simulink model "THSDemo"  (R2023a)
settings: Solver=ode4  StartTime=210  StopTime=260  FixedStep=0.002  RelTol=1e-3
InitFcn:
  |  T_c = 0.002;
undefined symbols (not defined in the file or in its folder): DiscIntNeverNeededParam, Discrete, magnitude, Time
libraries: simulink x23, simulink_extras x8, sharedtransform x3, ctrlSharedLib x2, aerolibconvert2 x1, aerolibtransform2 x1, dspstat3 x1, dspsolvers x1
(part 2 of 2)

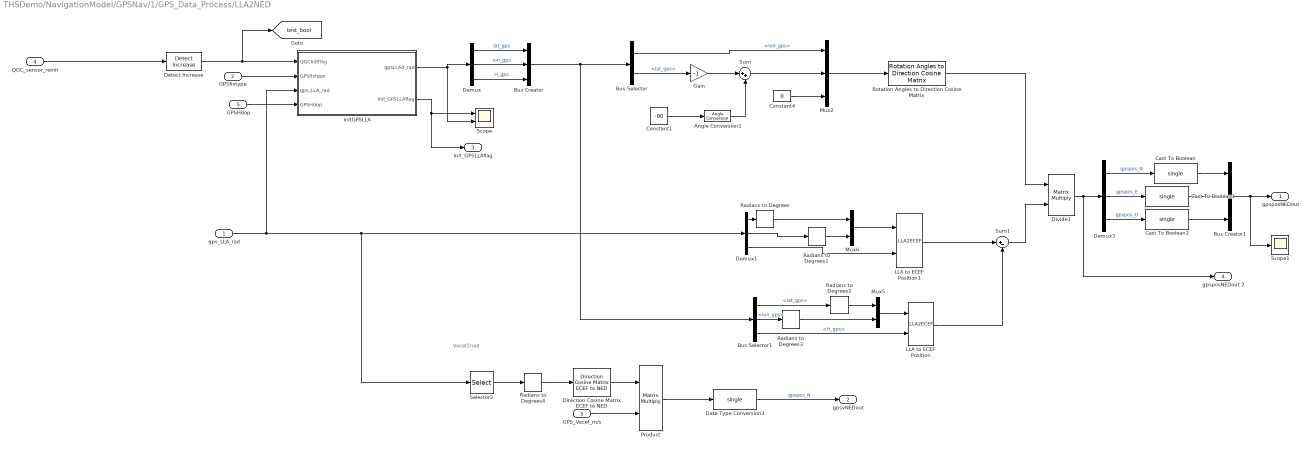
== system THSDemo/NavigationModel/GPSNav/1/GPS_Data_Process/LLA2NED ==
  note: Vecef2ned
  gps_LLA_rad : Inport
  GPSfixtype : Inport  Port=2
  GPS_Vecef_m/s : Inport  Port=3
  QGC_sensor_reinit : Inport  Port=4
  GPSHdop : Inport  Port=5
  Angle Conversion1 : aerolibconvert2/Angle Conversion  IU=deg  OU=rad
  Bus Creator : BusCreator  Inputs=3
  Bus Creator1 : BusCreator  Inputs=3
  Bus Selector : BusSelector  OutputSignals=lon_gps,lat_gps
  Bus Selector1 : BusSelector  OutputSignals=lat_gps,lon_gps,H_gps
  Cast To Boolean : DataTypeConversion  OutDataTypeStr=single  SaturateOnIntegerOverflow=off  RndMeth=Floor
  Cast To Boolean1 : DataTypeConversion  OutDataTypeStr=single  SaturateOnIntegerOverflow=off  RndMeth=Floor
  Cast To Boolean2 : DataTypeConversion  OutDataTypeStr=single  SaturateOnIntegerOverflow=off  RndMeth=Floor
  Constant1 : Constant  Value=-90
  Constant4 : Constant  Value=0
  Data Type Conversion3 : DataTypeConversion  OutDataTypeStr=single  SaturateOnIntegerOverflow=off  RndMeth=Floor
  Demux : Demux  Outputs=3
  Demux1 : Demux  Outputs=3
  Demux3 : Demux  Outputs=3
  Detect Increase : simulink/Logic and Bit Operations/Detect Increase  vinit=0.0  OutDataTypeStr=boolean
  Direction Cosine Matrix ECEF to NED : aerolibtransform2/Direction Cosine Matrix ECEF to NED
  Divide1 : Product  Inputs=**  Multiplication=Matrix(*)
  Gain : Gain  Gain=-1
  LLA to ECEF Position : LLA2ECEF  R=6378137
  LLA to ECEF Position1 : LLA2ECEF  R=6378137
  Mux2 : Mux  Inputs=3
  Mux5 : Mux  Inputs=2
  Mux6 : Mux  Inputs=2
  Product : Product  Multiplication=Matrix(*)
  Radians to Degrees{,1..4} (5 alike) : simulink_extras/Transformations/Radians to Degrees
  Rotation Angles to Direction Cosine Matrix : sharedtransform/Rotation Angles to Direction Cosine Matrix  rotationOrder=ZYX  aMode=aMode
  Scope : Scope  NumInputPorts=2
  Scope1 : Scope
  Selector2 : Selector  InputPortWidth=3  IndexOptions=Index vector (dialog)  Indices=[1 2]  OutputSizes=1
  Sum : Sum  Inputs=|++
  Sum1 : Sum  Inputs=|+-
  initGPSLLA : MATLAB Function  TreatAsAtomicUnit=on
  "gpsposNEDout " : Outport
  gpsvNEDout : Outport  Port=2
  init_GPSLLAflag : Outport  Port=3
  gpsposNEDout 2 : Outport  Port=4
  tag scope: test_bool=global
  wires:
  GPSfixtype/1 -> initGPSLLA/2(GPSfixtype)
  Bus Creator1/1 -> Scope1/1, "gpsposNEDout "/1
  Demux3/3 -> Cast To Boolean2/1  "gpspos_D"
  Demux3/2 -> Cast To Boolean1/1  "gpspos_E"
  Demux3/1 -> Cast To Boolean/1  "gpspos_N"
  Bus Creator/1 -> Bus Selector/1, Bus Selector1/1
  Demux/3 -> Bus Creator/3  "H_gps"
  Demux/2 -> Bus Creator/2  "lon_gps"
  Demux/1 -> Bus Creator/1  "lat_gps"
  Demux1/3 -> LLA to ECEF Position1/2
  Mux6/1 -> LLA to ECEF Position1/1
  Mux5/1 -> LLA to ECEF Position/1
  Gain/1 -> Sum/1
  LLA to ECEF Position1/1 -> Sum1/1
  Constant4/1 -> Mux2/3
  Sum1/1 -> Divide1/2
  Divide1/1 -> gpsposNEDout 2/1, Demux3/1
  Demux1/1 -> Radians to Degrees/1
  Mux2/1 -> Rotation Angles to Direction Cosine Matrix/1
  Rotation Angles to Direction Cosine Matrix/1 -> Divide1/1
  Constant1/1 -> Angle Conversion1/1
  LLA to ECEF Position/1 -> Sum1/2
  Demux1/2 -> Radians to Degrees1/1
  Sum/1 -> Mux2/2
  Bus Selector/2 -> Gain/1  "<lat_gps>"
  Bus Selector/1 -> Mux2/1  "<lon_gps>"
  Bus Selector1/1 -> Radians to Degrees2/1  "<lat_gps>"
  Bus Selector1/2 -> Radians to Degrees3/1  "<lon_gps>"
  Bus Selector1/3 -> LLA to ECEF Position/2  "<H_gps>"
  gps_LLA_rad/1 -> initGPSLLA/3(gps_LLA_rad), Selector2/1, Demux1/1
  Radians to Degrees/1 -> Mux6/1
  Radians to Degrees1/1 -> Mux6/2
  Angle Conversion1/1 -> Sum/2
  Radians to Degrees2/1 -> Mux5/1
  Radians to Degrees3/1 -> Mux5/2
  GPS_Vecef_m/s/1 -> Product/2
  Direction Cosine Matrix ECEF to NED/1 -> Product/1
  Selector2/1 -> Radians to Degrees4/1
  Radians to Degrees4/1 -> Direction Cosine Matrix ECEF to NED/1
  Data Type Conversion3/1 -> gpsvNEDout/1  "gpspos_N"
  Detect Increase/1 -> [test_bool], initGPSLLA/1(QGCinitflag)
  initGPSLLA/1(gpsLLA0_rad) -> Demux/1, Scope/2
  initGPSLLA/2(init_GPSLLAflag) -> init_GPSLLAflag/1, Scope/1
  GPSHdop/1 -> initGPSLLA/4(GPSHdop)
  Cast To Boolean/1 -> Bus Creator1/1
  Cast To Boolean1/1 -> Bus Creator1/2
  Cast To Boolean2/1 -> Bus Creator1/3
  QGC_sensor_reinit/1 -> Detect Increase/1
  Product/1 -> Data Type Conversion3/1

== system THSDemo/NavigationModel/GPSNav/1/GPS_Data_Process/TD_baro ==
  H_baro : Inport
  Constant1 : Constant  Value=0.002  OutDataTypeStr=double
  Constant3 : Constant  Value=0.23  OutDataTypeStr=double
  Constant4 : Constant  Value=900  OutDataTypeStr=single
  Data Type Conversion : DataTypeConversion  OutDataTypeStr=single  SaturateOnIntegerOverflow=off  RndMeth=Floor
  Data Type Conversion1 : DataTypeConversion  OutDataTypeStr=single  SaturateOnIntegerOverflow=off  RndMeth=Floor
  Data Type Conversion5 : DataTypeConversion  OutDataTypeStr=single  SaturateOnIntegerOverflow=off  RndMeth=Floor
  Delay1 : Delay  DelayLength=1  InitialConditionSource=Input port
      settings: InputPortMap=u0,p4
  MATLAB Function2 : MATLAB Function  TreatAsAtomicUnit=on
  Memory : Memory  InheritSampleTime=on
  Scope : Scope  NumInputPorts=3
  vH_baro_TD : Outport
  H_baro_TD : Outport  Port=2
  wires:
  Delay1/1 -> H_baro_TD/1, Scope/3, MATLAB Function2/3("u1 ")
  H_baro/1 -> Data Type Conversion5/1
  Memory/1 -> MATLAB Function2/4("u2 "), vH_baro_TD/1, Scope/2
  Constant3/1 -> Data Type Conversion1/1
  Constant4/1 -> MATLAB Function2/6(r)
  MATLAB Function2/1(u1) -> Delay1/1
  MATLAB Function2/2(u2) -> Memory/1
  Data Type Conversion5/1 -> Scope/1, Delay1/2, MATLAB Function2/2(u0)
  Constant1/1 -> Data Type Conversion/1
  Data Type Conversion/1 -> MATLAB Function2/1(T)
  Data Type Conversion1/1 -> MATLAB Function2/5(h)

== system THSDemo/NavigationModel/GPSNav/1/GPS_Data_Process/TD_baro1 ==
  H_baro : Inport
  Constant1 : Constant  Value=0.002  OutDataTypeStr=double
  Constant3 : Constant  Value=0.23  OutDataTypeStr=double
  Constant4 : Constant  Value=900  OutDataTypeStr=single
  Data Type Conversion : DataTypeConversion  OutDataTypeStr=single  SaturateOnIntegerOverflow=off  RndMeth=Floor
  Data Type Conversion1 : DataTypeConversion  OutDataTypeStr=single  SaturateOnIntegerOverflow=off  RndMeth=Floor
  Data Type Conversion5 : DataTypeConversion  OutDataTypeStr=single  SaturateOnIntegerOverflow=off  RndMeth=Floor
  Delay1 : Delay  DelayLength=1  InitialConditionSource=Input port
      settings: InputPortMap=u0,p4
  MATLAB Function2 : MATLAB Function  TreatAsAtomicUnit=on
  Memory : Memory  InheritSampleTime=on
  Scope : Scope  NumInputPorts=3
  vH_baro_TD : Outport
  H_baro_TD : Outport  Port=2
  wires:
  Data Type Conversion5/1 -> MATLAB Function2/2(u0), Delay1/2, Scope/1
  MATLAB Function2/2(u2) -> Memory/1
  MATLAB Function2/1(u1) -> Delay1/1
  Constant4/1 -> MATLAB Function2/6(r)
  Constant1/1 -> Data Type Conversion/1
  Constant3/1 -> Data Type Conversion1/1
  Memory/1 -> Scope/2, vH_baro_TD/1, MATLAB Function2/4("u2 ")
  H_baro/1 -> Data Type Conversion5/1
  Delay1/1 -> MATLAB Function2/3("u1 "), Scope/3, H_baro_TD/1
  Data Type Conversion/1 -> MATLAB Function2/1(T)
  Data Type Conversion1/1 -> MATLAB Function2/5(h)

== system THSDemo/NavigationModel/GPSNav/1/GPS_Data_Process/heading_GPS ==
  Vned : Inport
  Atan2 : Trigonometry  Operator=atan2
  Compare To Constant : simulink/Logic and Bit Operations/Compare To Constant  relop=>  const=0.8  OutDataTypeStr=boolean
  Data Type Conversion : DataTypeConversion  OutDataTypeStr=double  SaturateOnIntegerOverflow=off  RndMeth=Floor
  Math Function : Math  Operator=magnitude^2  SignedPower=on
  Moving Average1 : dspstat3/Moving Average  Commented=on  Method=Sliding window  ForgettingFactorPort=off  SpecifyWindowLength=on  WindowLength=10  OverlapLength=9  AllowArbitraryInputLength=off  ForgettingFactor=0.9  SimulateUsing=Code generation
  Rate Transition : RateTransition  OutPortSampleTime=1
  Scope : Scope  NumInputPorts=2
  Scope1 : Scope
  Selector2 : Selector  InputPortWidth=3  IndexOptions=Index vector (dialog)  Indices=[2]  OutputSizes=1
  Selector3 : Selector  InputPortWidth=3  IndexOptions=Index vector (dialog)  Indices=[1]  OutputSizes=1
  Selector4 : Selector  InputPortWidth=3  IndexOptions=Index vector (dialog)  Indices=[1 2]  OutputSizes=1
  Sqrt : Sqrt
  Sum of Elements : Sum  Inputs=+
  heading_GPS_rad : Outport
  heading_GPS_valid : Outport  Port=2
  wires:
  Selector2/1 -> Atan2/1
  Math Function/1 -> Sum of Elements/1
  Vned/1 -> Selector2/1, Selector4/1, Selector3/1
  Selector3/1 -> Atan2/2
  Sum of Elements/1 -> Sqrt/1
  Selector4/1 -> Math Function/1
  Sqrt/1 -> Data Type Conversion/1
  Compare To Constant/1 -> Scope1/1, heading_GPS_valid/1
  Rate Transition/1 -> Scope/1, Scope/2, heading_GPS_rad/1
  Atan2/1 -> Rate Transition/1
  Data Type Conversion/1 -> Compare To Constant/1

== system THSDemo/NavigationModel/GPSNav/1/Translation_estimate/Subsystem ==
  vxy : Inport
  pxy_GPS : Inport  Port=2
  GPSv_enable : Inport  Port=3
  QGC_init : Inport  Port=4
  DOP : Inport  Port=5
  Add : Sum  Inputs=+-
  Add1 : Sum  Inputs=++-
  Compare To Constant : simulink/Logic and Bit Operations/Compare To Constant  relop=<=  const=3  OutDataTypeStr=boolean
  Delay : Delay  DelayLength=1  InitialCondition=[0;0;]  ExternalReset=Rising
      settings: InputPortMap=u0,r5
  Detect Change : simulink/Logic and Bit Operations/Detect Change  vinit=0  OutDataTypeStr=boolean
  Gain : Gain  Gain=0.002
  Kalman Filter : ctrlSharedLib/Kalman Filter  TimeDomain=Discrete-Time  UseCurrentEstimator=on  ModelSource=Individual A, B, C, D matrices  ModelSourceVariable=ss(0.95,1,1,0,1)  A=[0.1,0;0,0.1]  B=eye(2)  C=eye(2)  D=0  NumberOfStates=1  NumberOfInputs=1  NumberOfOutputs=1  InitialEstimateSource=Dialog  X0=0  P0=10  UseK=off  UseGH=off  NumberOfProcessNoiseInputs=1  G=1  TimeInvariantG=on  H=0  TimeInvariantH=on  Q=diag([0.1;0.1])  TimeInvariantQ=on  R=diag([0.8;0.8])  TimeInvariantR=on  N=0  TimeInvariantN=on  AddInputPort=off  AddEnablePort=on  ExternalReset=Rising  OutputEstimatedY=off  OutputP=off  Ts=-1
  Logical Operator : Logic  AllPortsSameDT=off  OutDataTypeStr=boolean
  Memory : Memory
  Product : Product  OutDataTypeStr=double
  QGC_init1 : InportShadow  Port=4
  Rate Transition1 : RateTransition  OutPortSampleTime=0.002
  Rate Transition2 : RateTransition  OutPortSampleTime=0.002
  Rate Transition3 : RateTransition  OutPortSampleTime=0.002
  Scope7 : Scope
  Selector : Selector  InputPortWidth=2  IndexOptions=Index vector (dialog)  Indices=[1]  OutputSizes=1
  pxy_est : Outport
  wires:
  Gain/1 -> Add1/1
  Delay/1 -> Add1/2
  Kalman Filter/1 -> Product/1
  pxy_GPS/1 -> Selector/1, Add/2
  Selector/1 -> Detect Change/1
  Product/1 -> Memory/1
  Logical Operator/1 -> Product/2, Rate Transition2/1
  Rate Transition2/1 -> Scope7/1, Kalman Filter/2
  Rate Transition1/1 -> Kalman Filter/1
  Memory/1 -> Add1/3
  Add/1 -> Rate Transition1/1
  vxy/1 -> Gain/1
  Add1/1 -> Add/1, Delay/1, pxy_est/1
  QGC_init/1 -> Rate Transition3/1
  Rate Transition3/1 -> Kalman Filter/3
  DOP/1 -> Compare To Constant/1
  Compare To Constant/1 -> Logical Operator/2
  QGC_init1/1 -> Delay/2
  GPSv_enable/1 -> Logical Operator/1

== system THSDemo/NavigationModel/GPSNav/1/Translation_estimate/Subsystem2 ==
  axy : Inport
  vxy_GPS : Inport  Port=2
  QGC_init : Inport  Port=3
  DOP : Inport  Port=4
  Add : Sum  Inputs=+-
  Add1 : Sum  Inputs=++-
  Compare To Constant : simulink/Logic and Bit Operations/Compare To Constant  relop=<=  const=3  OutDataTypeStr=boolean
  Delay : Delay  DelayLength=1  ExternalReset=Rising
      settings: InputPortMap=u0,r5
  Detect Change : simulink/Logic and Bit Operations/Detect Change  vinit=0  OutDataTypeStr=boolean
  Gain : Gain  Gain=0.002
  Kalman Filter : ctrlSharedLib/Kalman Filter  TimeDomain=Discrete-Time  UseCurrentEstimator=on  ModelSource=Individual A, B, C, D matrices  ModelSourceVariable=ss(0.95,1,1,0,1)  A=[0.6,0;0,0.6]  B=eye(2)  C=eye(2)  D=0  NumberOfStates=1  NumberOfInputs=1  NumberOfOutputs=1  InitialEstimateSource=Dialog  X0=0  P0=10  UseK=off  UseGH=off  NumberOfProcessNoiseInputs=1  G=1  TimeInvariantG=on  H=0  TimeInvariantH=on  Q=diag([0.1;0.1])  TimeInvariantQ=on  R=diag([0.6;0.6])  TimeInvariantR=on  N=0  TimeInvariantN=on  AddInputPort=off  AddEnablePort=on  ExternalReset=Rising  OutputEstimatedY=off  OutputP=off  Ts=-1
  Logical Operator : Logic  AllPortsSameDT=off  OutDataTypeStr=boolean
  Memory : Memory
  Product : Product  OutDataTypeStr=double
  Rate Transition1 : RateTransition  OutPortSampleTime=0.002
  Rate Transition2 : RateTransition  OutPortSampleTime=0.002
  Rate Transition3 : RateTransition  OutPortSampleTime=0.002
  Scope : Scope  NumInputPorts=2
  Scope7 : Scope
  Selector : Selector  InputPortWidth=2  IndexOptions=Index vector (dialog)  Indices=[1]  OutputSizes=1
  vxy_est : Outport
  GPSv_enable : Outport  Port=2
  wires:
  Compare To Constant/1 -> Logical Operator/2
  DOP/1 -> Compare To Constant/1
  Detect Change/1 -> Logical Operator/1
  Rate Transition3/1 -> Kalman Filter/3
  QGC_init/1 -> Delay/2, Rate Transition3/1
  Add1/1 -> Delay/1, vxy_est/1, Scope/1, Add/1
  Add/1 -> Rate Transition1/1
  Memory/1 -> Add1/3
  Rate Transition1/1 -> Kalman Filter/1
  Rate Transition2/1 -> Scope7/1, Kalman Filter/2
  Logical Operator/1 -> GPSv_enable/1, Rate Transition2/1, Product/2
  Product/1 -> Memory/1
  Selector/1 -> Detect Change/1
  vxy_GPS/1 -> Selector/1, Add/2, Scope/2
  Kalman Filter/1 -> Product/1
  Gain/1 -> Add1/1
  axy/1 -> Gain/1
  Delay/1 -> Add1/2

== system THSDemo/NavigationModel/GPSNav/1/Translation_estimate/V_Horizontal_estimation1 ==
  note: 0530改：
      | 加入GPStype限制
  An : Inport
  vn_gps : Inport  Port=2
  ve_gps : Inport  Port=3
  fixtype_gps : Inport  Port=4
  QGC_init : Inport  Port=5
  Add : Sum  Inputs=+-
  Compare To Constant : simulink/Logic and Bit Operations/Compare To Constant  relop=>=  const=3  OutDataTypeStr=boolean
  Delay : Delay  DelayLength=1
  Detect Change : simulink/Logic and Bit Operations/Detect Change  vinit=0  OutDataTypeStr=boolean
  Integrator_V_Horizontal : Subsystem
  Logical Operator : Logic  AllPortsSameDT=off  OutDataTypeStr=boolean
  Mux : Mux  Inputs=2
  Rxy_kalman filter1 : Subsystem  mask{F=diag([-0.1,-0.1,-0.002,-0.002]), H=[1,0,-1,0;0,1,0,-1], Q=diag([1,1,0.1,0.1]), R=diag([0.001,0.001]), P0=diag([0.8,0.8,0.2,0.2])}
      mask prompts: F "状态转移矩阵：F"; H "观测转移矩阵：H"; Q "预测噪声协方差矩阵：Q"; R "量测噪声协方差矩阵：R"; P0 "初始协方差矩阵：P0"
      mask DialogControl DescTextVar Prompt: Kalman Filter
  Scope : Scope  NumInputPorts=2
  Scope1 : Scope
  Selector : Selector  InputPortWidth=4  IndexOptions=Index vector (dialog)  Indices=[1 2]  OutputSizes=1
  vxy_estimout : Outport
  GPS_v_enable : Outport  Port=2
  wires:
  QGC_init/1 -> Integrator_V_Horizontal/3(QGC_init)
  Delay/1 -> Selector/1, Rxy_kalman filter1/1(X)
  Selector/1 -> Integrator_V_Horizontal/2(dv)
  vn_gps/1 -> Integrator_V_Horizontal/4(vn_gps), Mux/1, Detect Change/1
  Mux/1 -> Scope/2, Add/2
  ve_gps/1 -> Integrator_V_Horizontal/5(ve_gps), Mux/2
  Rxy_kalman filter1/1(XOut) -> Delay/1
  Integrator_V_Horizontal/1(V_n&e) -> Add/1, vxy_estimout/1, Scope/1
  Add/1 -> Rxy_kalman filter1/2(Z)
  An/1 -> Integrator_V_Horizontal/1(An)
  fixtype_gps/1 -> Compare To Constant/1
  Detect Change/1 -> Logical Operator/1
  Compare To Constant/1 -> Logical Operator/2, Scope1/1, GPS_v_enable/1, Rxy_kalman filter1/3(Enable), Integrator_V_Horizontal/6(GPSenable)

== system THSDemo/NavigationModel/GPSNav/1/Translation_estimate/translate to N ==
  Cbn : Inport
  accl_ned : Inport  Port=2
  Product : Product  Multiplication=Matrix(*)
  Selector : Selector  InputPortWidth=3  IndexOptions=Index vector (dialog)  Indices=[1 2]  OutputSizes=1
  accel_Horizontal_predict : Outport
  wires:
  Selector/1 -> accel_Horizontal_predict/1
  Product/1 -> Selector/1
  Cbn/1 -> Product/1
  accl_ned/1 -> Product/2

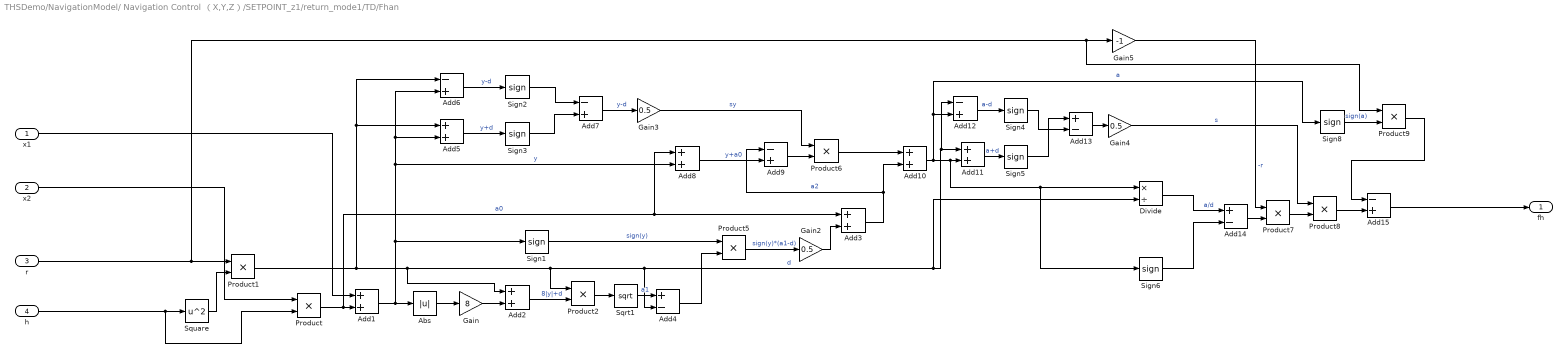
== system THSDemo/NavigationModel/ Navigation Control （X,Y,Z）/SETPOINT_z1/return_mode1/TD/Fhan ==
  x1 : Inport
  x2 : Inport  Port=2
  r : Inport  Port=3
  h : Inport  Port=4
  Abs : Abs  SaturateOnIntegerOverflow=off
  Add{1..3,5,8,10..11} (7 alike) : Sum
  Add{6..7,9,12,15} (5 alike) : Sum  Inputs=-+
  Add13 : Sum  Inputs=+-
  Add14 : Sum  Inputs=+-
  Add4 : Sum  Inputs=+-
  Divide : Product  Inputs=*/
  Gain : Gain  Gain=8
  Gain2 : Gain  Gain=0.5
  Gain3 : Gain  Gain=0.5
  Gain4 : Gain  Gain=0.5
  Gain5 : Gain  Gain=-1
  Product{,1..2,5..9} (8 alike) : Product
  Sign{1..6,8} (7 alike) : Signum
  Sqrt1 : Sqrt
  Square : Math  Operator=square  SignedPower=on
  fh : Outport
  wires:
  Add1/1 -> Add8/2, Add6/2, Add5/2, Sign1/1, Abs/1  "y"
  Product1/1 -> Add6/1, Add5/1, Divide/2, Add12/1, Add11/1, Add4/2, Product2/1, Add2/1  "d"
  Add5/1 -> Sign3/1  "y+d"
  Sign4/1 -> Add13/2
  Add9/1 -> Product6/2
  Product5/1 -> Gain2/1  "sign(y)*(a1-d)"
  Gain3/1 -> Product6/1  "sy"
  Product/1 -> Add8/1, Add3/1, Add1/2  "a0"
  Product6/1 -> Add10/1
  Add7/1 -> Gain3/1  "y-d"
  Sign8/1 -> Product9/2  "sign(a)"
  Sign3/1 -> Add7/2
  Add2/1 -> Product2/2  "8|y|+d"
  r/1 -> Product9/1, Gain5/1, Product1/1
  Add10/1 -> Sign6/1, Divide/1, Add11/2, Add12/2, Sign8/1  "a"
  Product2/1 -> Sqrt1/1
  Sign5/1 -> Add13/1
  Abs/1 -> Gain/1
  Divide/1 -> Add14/1  "a/d"
  Gain2/1 -> Add3/2
  Gain/1 -> Add2/2
  Add13/1 -> Gain4/1
  Add14/1 -> Product7/2
  Add3/1 -> Add10/2, Add9/1  "a2"
  Add12/1 -> Sign4/1  "a-d"
  Gain4/1 -> Product8/1  "s"
  Product8/1 -> Add15/2
  h/1 -> Product/2, Square/1
  Square/1 -> Product1/2
  Add8/1 -> Add9/2  "y+a0"
  Sign6/1 -> Add14/2
  Add11/1 -> Sign5/1  "a+d"
  Sign2/1 -> Add7/1
  Sqrt1/1 -> Add4/1  "a1"
  Product9/1 -> Add15/1
  Add4/1 -> Product5/2
  Add6/1 -> Sign2/1  "y-d"
  Sign1/1 -> Product5/1  "sign(y)"
  Product7/1 -> Product8/2
  Gain5/1 -> Product7/1  "-r"
  x1/1 -> Add1/1
  x2/1 -> Product/1
  Add15/1 -> fh/1

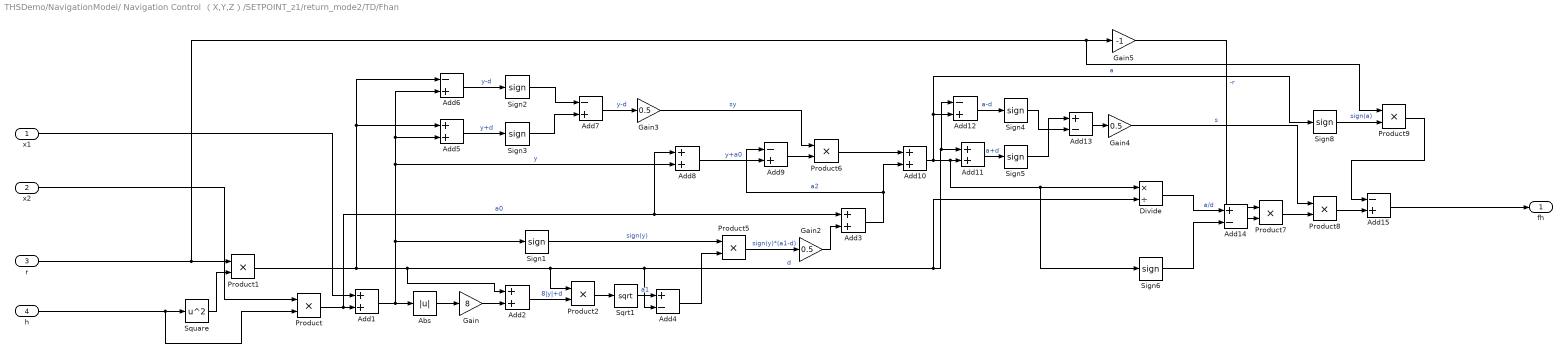
== system THSDemo/NavigationModel/ Navigation Control （X,Y,Z）/SETPOINT_z1/return_mode2/TD/Fhan ==
  x1 : Inport
  x2 : Inport  Port=2
  r : Inport  Port=3
  h : Inport  Port=4
  Abs : Abs  SaturateOnIntegerOverflow=off
  Add{1..3,5,8,10..11} (7 alike) : Sum
  Add{6..7,9,12,15} (5 alike) : Sum  Inputs=-+
  Add13 : Sum  Inputs=+-
  Add14 : Sum  Inputs=+-
  Add4 : Sum  Inputs=+-
  Divide : Product  Inputs=*/
  Gain : Gain  Gain=8
  Gain2 : Gain  Gain=0.5
  Gain3 : Gain  Gain=0.5
  Gain4 : Gain  Gain=0.5
  Gain5 : Gain  Gain=-1
  Product{,1..2,5..9} (8 alike) : Product
  Sign{1..6,8} (7 alike) : Signum
  Sqrt1 : Sqrt
  Square : Math  Operator=square  SignedPower=on
  fh : Outport
  wires:
  Add15/1 -> fh/1
  x2/1 -> Product/1
  x1/1 -> Add1/1
  Gain5/1 -> Product7/1  "-r"
  Product7/1 -> Product8/2
  Sign1/1 -> Product5/1  "sign(y)"
  Add6/1 -> Sign2/1  "y-d"
  Add4/1 -> Product5/2
  Product9/1 -> Add15/1
  Sqrt1/1 -> Add4/1  "a1"
  Sign2/1 -> Add7/1
  Add11/1 -> Sign5/1  "a+d"
  Sign6/1 -> Add14/2
  Add8/1 -> Add9/2  "y+a0"
  Square/1 -> Product1/2
  h/1 -> Square/1, Product/2
  Product8/1 -> Add15/2
  Gain4/1 -> Product8/1  "s"
  Add12/1 -> Sign4/1  "a-d"
  Add3/1 -> Add9/1, Add10/2  "a2"
  Add14/1 -> Product7/2
  Add13/1 -> Gain4/1
  Gain/1 -> Add2/2
  Gain2/1 -> Add3/2
  Divide/1 -> Add14/1  "a/d"
  Abs/1 -> Gain/1
  Sign5/1 -> Add13/1
  Product2/1 -> Sqrt1/1
  Add10/1 -> Sign8/1, Add12/2, Add11/2, Divide/1, Sign6/1  "a"
  r/1 -> Product1/1, Gain5/1, Product9/1
  Add2/1 -> Product2/2  "8|y|+d"
  Sign3/1 -> Add7/2
  Sign8/1 -> Product9/2  "sign(a)"
  Add7/1 -> Gain3/1  "y-d"
  Product6/1 -> Add10/1
  Product/1 -> Add1/2, Add3/1, Add8/1  "a0"
  Gain3/1 -> Product6/1  "sy"
  Product5/1 -> Gain2/1  "sign(y)*(a1-d)"
  Add9/1 -> Product6/2
  Sign4/1 -> Add13/2
  Add5/1 -> Sign3/1  "y+d"
  Product1/1 -> Add2/1, Product2/1, Add4/2, Add11/1, Add12/1, Divide/2, Add5/1, Add6/1  "d"
  Add1/1 -> Abs/1, Sign1/1, Add5/2, Add6/2, Add8/2  "y"

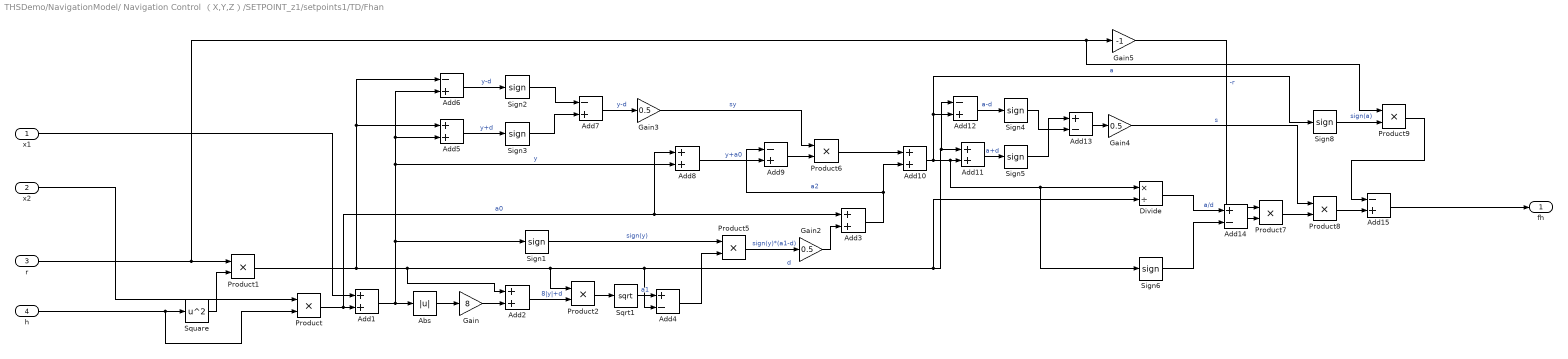
== system THSDemo/NavigationModel/ Navigation Control （X,Y,Z）/SETPOINT_z1/setpoints1/TD/Fhan ==
  x1 : Inport
  x2 : Inport  Port=2
  r : Inport  Port=3
  h : Inport  Port=4
  Abs : Abs  SaturateOnIntegerOverflow=off
  Add{1..3,5,8,10..11} (7 alike) : Sum
  Add{6..7,9,12,15} (5 alike) : Sum  Inputs=-+
  Add13 : Sum  Inputs=+-
  Add14 : Sum  Inputs=+-
  Add4 : Sum  Inputs=+-
  Divide : Product  Inputs=*/
  Gain : Gain  Gain=8
  Gain2 : Gain  Gain=0.5
  Gain3 : Gain  Gain=0.5
  Gain4 : Gain  Gain=0.5
  Gain5 : Gain  Gain=-1
  Product{,1..2,5..9} (8 alike) : Product
  Sign{1..6,8} (7 alike) : Signum
  Sqrt1 : Sqrt
  Square : Math  Operator=square  SignedPower=on
  fh : Outport
  wires:
  Add1/1 -> Add8/2, Add6/2, Add5/2, Sign1/1, Abs/1  "y"
  Product1/1 -> Add6/1, Add5/1, Divide/2, Add12/1, Add11/1, Add4/2, Product2/1, Add2/1  "d"
  Add5/1 -> Sign3/1  "y+d"
  Sign4/1 -> Add13/2
  Add9/1 -> Product6/2
  Product5/1 -> Gain2/1  "sign(y)*(a1-d)"
  Gain3/1 -> Product6/1  "sy"
  Product/1 -> Add8/1, Add3/1, Add1/2  "a0"
  Product6/1 -> Add10/1
  Add7/1 -> Gain3/1  "y-d"
  Sign8/1 -> Product9/2  "sign(a)"
  Sign3/1 -> Add7/2
  Add2/1 -> Product2/2  "8|y|+d"
  r/1 -> Product9/1, Gain5/1, Product1/1
  Add10/1 -> Sign6/1, Divide/1, Add11/2, Add12/2, Sign8/1  "a"
  Product2/1 -> Sqrt1/1
  Sign5/1 -> Add13/1
  Abs/1 -> Gain/1
  Divide/1 -> Add14/1  "a/d"
  Gain2/1 -> Add3/2
  Gain/1 -> Add2/2
  Add13/1 -> Gain4/1
  Add14/1 -> Product7/2
  Add3/1 -> Add10/2, Add9/1  "a2"
  Add12/1 -> Sign4/1  "a-d"
  Gain4/1 -> Product8/1  "s"
  Product8/1 -> Add15/2
  h/1 -> Product/2, Square/1
  Square/1 -> Product1/2
  Add8/1 -> Add9/2  "y+a0"
  Sign6/1 -> Add14/2
  Add11/1 -> Sign5/1  "a+d"
  Sign2/1 -> Add7/1
  Sqrt1/1 -> Add4/1  "a1"
  Product9/1 -> Add15/1
  Add4/1 -> Product5/2
  Add6/1 -> Sign2/1  "y-d"
  Sign1/1 -> Product5/1  "sign(y)"
  Product7/1 -> Product8/2
  Gain5/1 -> Product7/1  "-r"
  x1/1 -> Add1/1
  x2/1 -> Product/1
  Add15/1 -> fh/1

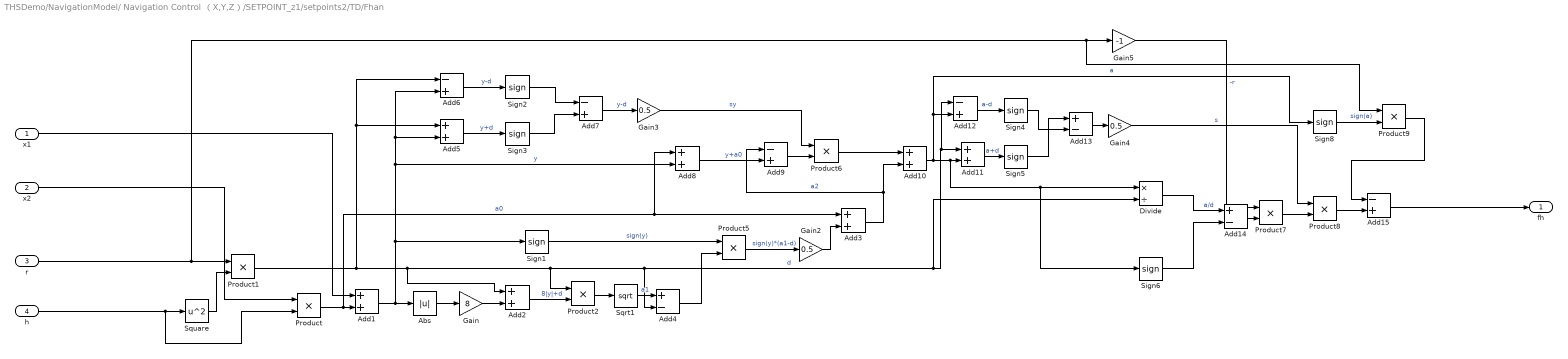
== system THSDemo/NavigationModel/ Navigation Control （X,Y,Z）/SETPOINT_z1/setpoints2/TD/Fhan ==
  x1 : Inport
  x2 : Inport  Port=2
  r : Inport  Port=3
  h : Inport  Port=4
  Abs : Abs  SaturateOnIntegerOverflow=off
  Add{1..3,5,8,10..11} (7 alike) : Sum
  Add{6..7,9,12,15} (5 alike) : Sum  Inputs=-+
  Add13 : Sum  Inputs=+-
  Add14 : Sum  Inputs=+-
  Add4 : Sum  Inputs=+-
  Divide : Product  Inputs=*/
  Gain : Gain  Gain=8
  Gain2 : Gain  Gain=0.5
  Gain3 : Gain  Gain=0.5
  Gain4 : Gain  Gain=0.5
  Gain5 : Gain  Gain=-1
  Product{,1..2,5..9} (8 alike) : Product
  Sign{1..6,8} (7 alike) : Signum
  Sqrt1 : Sqrt
  Square : Math  Operator=square  SignedPower=on
  fh : Outport
  wires:
  Add15/1 -> fh/1
  x2/1 -> Product/1
  x1/1 -> Add1/1
  Gain5/1 -> Product7/1  "-r"
  Product7/1 -> Product8/2
  Sign1/1 -> Product5/1  "sign(y)"
  Add6/1 -> Sign2/1  "y-d"
  Add4/1 -> Product5/2
  Product9/1 -> Add15/1
  Sqrt1/1 -> Add4/1  "a1"
  Sign2/1 -> Add7/1
  Add11/1 -> Sign5/1  "a+d"
  Sign6/1 -> Add14/2
  Add8/1 -> Add9/2  "y+a0"
  Square/1 -> Product1/2
  h/1 -> Square/1, Product/2
  Product8/1 -> Add15/2
  Gain4/1 -> Product8/1  "s"
  Add12/1 -> Sign4/1  "a-d"
  Add3/1 -> Add9/1, Add10/2  "a2"
  Add14/1 -> Product7/2
  Add13/1 -> Gain4/1
  Gain/1 -> Add2/2
  Gain2/1 -> Add3/2
  Divide/1 -> Add14/1  "a/d"
  Abs/1 -> Gain/1
  Sign5/1 -> Add13/1
  Product2/1 -> Sqrt1/1
  Add10/1 -> Sign8/1, Add12/2, Add11/2, Divide/1, Sign6/1  "a"
  r/1 -> Product1/1, Gain5/1, Product9/1
  Add2/1 -> Product2/2  "8|y|+d"
  Sign3/1 -> Add7/2
  Sign8/1 -> Product9/2  "sign(a)"
  Add7/1 -> Gain3/1  "y-d"
  Product6/1 -> Add10/1
  Product/1 -> Add1/2, Add3/1, Add8/1  "a0"
  Gain3/1 -> Product6/1  "sy"
  Product5/1 -> Gain2/1  "sign(y)*(a1-d)"
  Add9/1 -> Product6/2
  Sign4/1 -> Add13/2
  Add5/1 -> Sign3/1  "y+d"
  Product1/1 -> Add2/1, Product2/1, Add4/2, Add11/1, Add12/1, Divide/2, Add5/1, Add6/1  "d"
  Add1/1 -> Abs/1, Sign1/1, Add5/2, Add6/2, Add8/2  "y"

== system THSDemo/NavigationModel/GPSNav/1/Translation_estimate/V_Horizontal_estimation1/Integrator_V_Horizontal ==
  An : Inport
  dv : Inport  Port=2
  QGC_init : Inport  Port=3
  vn_gps : Inport  Port=4
  ve_gps : Inport  Port=5
  GPSenable : Inport  Port=6
  Delay : Delay  DelayLength=1  InitialConditionSource=Input port  ExternalReset=Rising
      settings: InputPortMap=u0,r5,p4
  Gain : Gain  Gain=0.8
  Gain2 : Gain  Gain=dt  SaturateOnIntegerOverflow=on  OutDataTypeStr=Inherit: Same as input  ParamDataTypeStr=Inherit: Same as input
  Mux : Mux  Inputs=2
  Product : Product
  Scope : Scope
  Sum : Sum  Inputs=|++-
  V_n&e : Outport
  wires:
  GPSenable/1 -> Product/2
  dv/1 -> Product/1
  An/1 -> Gain2/1
  Gain2/1 -> Sum/1
  Sum/1 -> V_n&e/1, Delay/1
  QGC_init/1 -> Delay/2
  vn_gps/1 -> Mux/1
  ve_gps/1 -> Mux/2
  Mux/1 -> Delay/3
  Delay/1 -> Sum/2
  Product/1 -> Gain/1
  Gain/1 -> Scope/1, Sum/3

== system THSDemo/NavigationModel/GPSNav/1/Translation_estimate/V_Horizontal_estimation1/Rxy_kalman filter1 ==
  X : Inport
  Z : Inport  Port=2
  Enable : Inport  Port=3
  Constant : Constant  Value=F  OutDataTypeStr=single
  Constant1 : Constant  Value=Q  OutDataTypeStr=single
  Constant2 : Constant  Value=R  OutDataTypeStr=single
  Constant3 : Constant  Value=P0  OutDataTypeStr=single
  Constant4 : Constant  Value=H  OutDataTypeStr=single
  Vxy kalman filter : Subsystem  TreatAsAtomicUnit=on
  XOut : Outport
  wires:
  Enable/1 -> Vxy kalman filter/9(Enable)
  Vxy kalman filter/1(XOut) -> XOut/1
  Constant1/1 -> Vxy kalman filter/5(Q)
  Constant4/1 -> Vxy kalman filter/4(H)
  Constant2/1 -> Vxy kalman filter/6(R)
  Constant3/1 -> Vxy kalman filter/8(P0)
  Z/1 -> Vxy kalman filter/1(Z)
  Constant/1 -> Vxy kalman filter/3(G), Vxy kalman filter/2(F)
  X/1 -> Vxy kalman filter/7(X)

== system THSDemo/NavigationModel/GPSNav/1/Translation_estimate/V_Horizontal_estimation1/Rxy_kalman filter1/Vxy kalman filter ==
  Z : Inport
  F : Inport  Port=2
  G : Inport  Port=3
  H : Inport  Port=4
  Q : Inport  Port=5
  R : Inport  Port=6
  X : Inport  Port=7
  P0 : Inport  Port=8
  Enable : Inport  Port=9
  Add1 : Sum
  Delay : Delay  DelayLength=1  InitialConditionSource=Input port
      settings: InputPortMap=u0,p4
  Gain4 : Gain  Gain=0.5
  Math Function : Math  Operator=transpose  SignedPower=on
  kalman : Subsystem
  XOut : Outport
  wires:
  P0/1 -> Delay/2
  Gain4/1 -> Delay/1
  Delay/1 -> kalman/7(P)
  Add1/1 -> Gain4/1
  Math Function/1 -> Add1/2
  Z/1 -> kalman/1(Z)
  F/1 -> kalman/2(F)
  G/1 -> kalman/3(G)
  H/1 -> kalman/4(H)
  Q/1 -> kalman/5(Q)
  R/1 -> kalman/6(R)
  X/1 -> kalman/8(X)
  kalman/1(POut) -> Math Function/1, Add1/1
  kalman/2(XOut) -> XOut/1
  Enable/1 -> kalman/9(Enable)

== system THSDemo/NavigationModel/GPSNav/1/Translation_estimate/V_Horizontal_estimation1/Rxy_kalman filter1/Vxy kalman filter/kalman ==
  note: Xk/k-1=FXk-1
      | Xk=Xk/k-1+K(Z-h(Xk/k-1))
      | K=Pk/k-1H(HPk/k-1H+Rk)-1
      | Pk/k-1=FPk-1F+GQG
      | Pk=(I-KH)Pk/k-1
  Z : Inport
  F : Inport  Port=2
  G : Inport  Port=3
  H : Inport  Port=4
  Q : Inport  Port=5
  R : Inport  Port=6
  P : Inport  Port=7
  X : Inport  Port=8
  Enable : Inport  Port=9
  Scope : Scope  NumInputPorts=2
  Subsystem : Subsystem
  Subsystem1 : Subsystem
  POut : Outport
  XOut : Outport  Port=2
  wires:
  X/1 -> [X]
  P/1 -> [P]
  Q/1 -> [Q]
  G/1 -> [G]
  F/1 -> [F]
  Z/1 -> [Z]
  [F] -> Subsystem/1(F)
  [G] -> Subsystem/2(G)
  [Q] -> Subsystem/3(Q)
  [X] -> Subsystem/4(X)
  [P] -> Subsystem/5(P)
  Subsystem/1(Xk_k_1) -> [Xk_k_1]
  Subsystem/2(Pk_k_1) -> [Pk_k_1]
  H/1 -> Subsystem1/3(H)
  R/1 -> Subsystem1/4(R)
  Subsystem1/1(POut) -> POut/1
  Subsystem1/2(XOut) -> XOut/1, Scope/2
  [Xk_k_1] -> Subsystem1/1(Xkk)
  [Pk_k_1] -> Subsystem1/2(Pkk)
  Enable/1 -> Subsystem1/Enable, Scope/1
  [Z] -> Subsystem1/5(Z)

== system THSDemo/NavigationModel/GPSNav/1/Translation_estimate/V_Horizontal_estimation1/Rxy_kalman filter1/Vxy kalman filter/kalman/Subsystem ==
  F : Inport
  G : Inport  Port=2
  Q : Inport  Port=3
  X : Inport  Port=4
  P : Inport  Port=5
  Add : Sum
  Math Function3 : Math  Operator=transpose  SignedPower=on
  Math Function4 : Math  Operator=transpose  SignedPower=on
  MatrixMultiply : Product  Multiplication=Matrix(*)
  MatrixMultiply1 : Product  Inputs=3  Multiplication=Matrix(*)
  MatrixMultiply8 : Product  Inputs=3  Multiplication=Matrix(*)
  Xk_k_1 : Outport
  Pk_k_1 : Outport  Port=2
  wires:
  Math Function4/1 -> MatrixMultiply8/3
  [Q] -> MatrixMultiply8/2
  MatrixMultiply/1 -> [Xk_k_1]
  MatrixMultiply1/1 -> Add/1
  [F] -> Math Function3/1
  Math Function3/1 -> MatrixMultiply1/3
  [P] -> MatrixMultiply1/2
  [F] -> MatrixMultiply1/1
  Add/1 -> [Pk_k_1]
  [G] -> MatrixMultiply8/1
  MatrixMultiply8/1 -> Add/2
  [X] -> MatrixMultiply/2
  [G] -> Math Function4/1
  [F] -> MatrixMultiply/1
  F/1 -> [F]
  G/1 -> [G]
  Q/1 -> [Q]
  X/1 -> [X]
  P/1 -> [P]
  [Xk_k_1] -> Xk_k_1/1
  [Pk_k_1] -> Pk_k_1/1

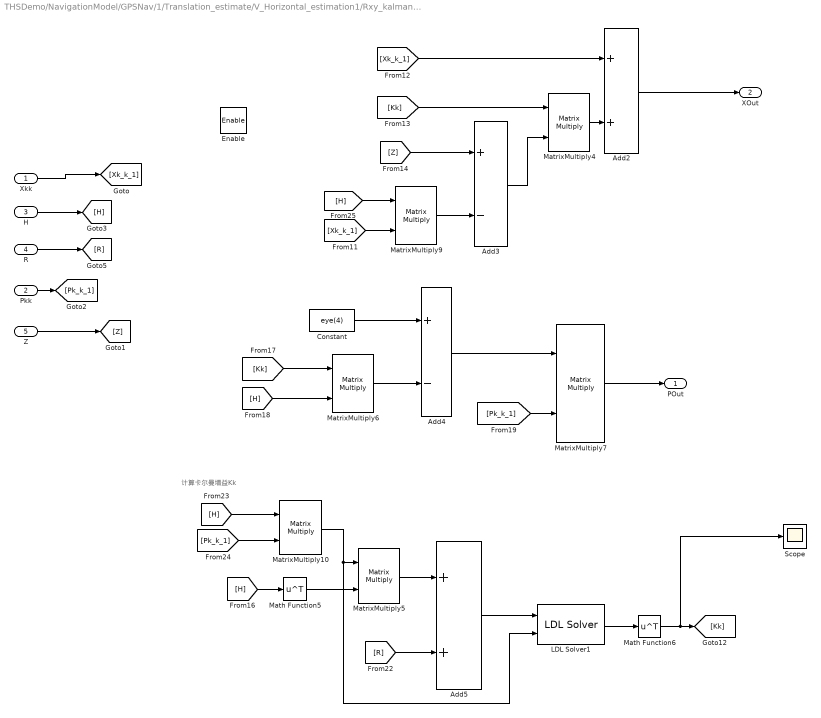
== system THSDemo/NavigationModel/GPSNav/1/Translation_estimate/V_Horizontal_estimation1/Rxy_kalman filter1/Vxy kalman filter/kalman/Subsystem1 ==
  note: 计算卡尔曼增益Kk
  Xkk : Inport
  Pkk : Inport  Port=2
  H : Inport  Port=3
  R : Inport  Port=4
  Z : Inport  Port=5
  Enable : EnablePort
  Add2 : Sum
  Add3 : Sum  Inputs=+-
  Add4 : Sum  Inputs=+-
  Add5 : Sum
  Constant : Constant  Value=eye(4)  OutDataTypeStr=single
  LDL Solver1 : dspsolvers/LDL Solver  errmode=Warning
      settings: RTWMemSecFuncInitTerm=Default  RTWMemSecFuncExecute=Default  RTWMemSecDataConstants=Default  RTWMemSecDataInternal=Default  RTWMemSecDataParameters=Default
  Math Function5 : Math  Operator=transpose  SignedPower=on
  Math Function6 : Math  Operator=transpose  SignedPower=on
  MatrixMultiply{4..7,9..10} (6 alike) : Product  Multiplication=Matrix(*)
  Scope : Scope
  POut : Outport
  XOut : Outport  Port=2
  wires:
  MatrixMultiply9/1 -> Add3/2
  MatrixMultiply7/1 -> POut/1
  [H] -> MatrixMultiply10/1
  Add3/1 -> MatrixMultiply4/2
  Math Function5/1 -> MatrixMultiply5/2
  Math Function6/1 -> Scope/1, [Kk]
  Add4/1 -> MatrixMultiply7/1
  MatrixMultiply4/1 -> Add2/2
  [Kk] -> MatrixMultiply4/1
  [Z] -> Add3/1
  MatrixMultiply10/1 -> MatrixMultiply5/1, LDL Solver1/2
  MatrixMultiply5/1 -> Add5/1
  LDL Solver1/1 -> Math Function6/1
  [H] -> Math Function5/1
  [Pk_k_1] -> MatrixMultiply10/2
  [R] -> Add5/2
  Constant/1 -> Add4/1
  [Kk] -> MatrixMultiply6/1
  [Xk_k_1] -> Add2/1
  [H] -> MatrixMultiply6/2
  [H] -> MatrixMultiply9/1
  [Xk_k_1] -> MatrixMultiply9/2
  [Pk_k_1] -> MatrixMultiply7/2
  R/1 -> [R]
  Add5/1 -> LDL Solver1/1
  MatrixMultiply6/1 -> Add4/2
  H/1 -> [H]
  Add2/1 -> XOut/1
  Xkk/1 -> [Xk_k_1]
  Z/1 -> [Z]
  Pkk/1 -> [Pk_k_1]

== stateflow chart THSDemo/NavigationModel/ Navigation Control （X,Y,Z）/SETPOINT_z1/setpoints1/Chart ==
  state Line
    en, du: flag_setpoint = 0;
  state Next
    en, du: flag_setpoint = 1;
  (default) -> Line
  Next -> Line : [dist < 1 ]
  Line -> Next : [dist > 0]
  data: dist input; flag_setpoint output

== stateflow chart THSDemo/NavigationModel/ Navigation Control （X,Y,Z）/SETPOINT_z1/setpoints2/Chart ==
  state Line
    en, du: flag_setpoint = 0;
  state Next
    en, du: flag_setpoint = 1;
  (default) -> Line
  Next -> Line : [dist < 1 ]
  Line -> Next : [dist > 0]
  data: dist input; flag_setpoint output

== matlab function THSDemo/NavigationModel/GPSNav/1/GPS_Data_Process/LLA2NED/initGPSLLA ==
  data: QGCinitflag input; gpsLLA0_rad output; GPSfixtype input; gps_LLA_rad input; init_GPSLLAflag output; GPSHdop input
function [gpsLLA0_rad,init_GPSLLAflag] = initGPSLLA0(QGCinitflag,GPSfixtype,gps_LLA_rad,GPSHdop)
    persistent initGPSLLAflag;
    persistent gpsLLA0;

    if isempty(initGPSLLAflag)
        initGPSLLAflag = 0;
    end
    if isempty(gpsLLA0)
        %初始GPS未进入定位状态，给定值
%          gpsLLA0 = [28.2/57.3;113/57.3;0];
        gpsLLA0 = zeros(3,1);
    end
    %if (initGPSLLAflag == 0 && GPSfixtype >= 3 && GPSHdop <= 2) || (QGCinitflag == 1 && GPSfixtype >= 3)
    if (initGPSLLAflag == 0 && GPSfixtype >= 1 && GPSHdop <= 5) || (QGCinitflag == 1 && GPSfixtype >= 1)
        % 当GPS第一次初始化位置时，当GPSfixtype >=1 时，自动初始化一次位置，initGPSLLAflag置1
        % 或者是利用QGCinitflag地面站重新修正，不过需要满足GPSfixtype>=1的条件
        gpsLLA0 = gps_LLA_rad;
        initGPSLLAflag = 1;
    end
    gpsLLA0_rad = gpsLLA0;
    init_GPSLLAflag = initGPSLLAflag;
end

== matlab function THSDemo/NavigationModel/GPSNav/1/GPS_Data_Process/TD_baro1/MATLAB Function2 ==
  data: T input single; u1 output; u0 input; u1 input single; u2 input single; h input single; r input single; u2 output
function [u1,u2]=diff_TD_2(T,u0,u1,u2,h,r)
    %init
    %T是信号周期，u0原始信号输入，u1跟踪原始信号，u2原始信号差分值，
    %h滤波因子（h=T时接近一阶差分）越大滤波好延迟大；r速度因子，越大跟踪的越快但是噪声放大；

x1=0; x2=0;
delta=0;
delta0=0;
y=0;
fabs_y=0;
a0=0;
a=0;
fst=0;

x1 = u1;
x2 = u2;
delta = r*h;
delta0 = delta*h;
y = x1 - u0 + h*x2;
fabs_y = abs(y);   
a0 = sqrt(delta*delta + 8 * r*fabs_y);

if (fabs_y <= delta0)
	a = x2 + y / h;
else
    a = x2 + 0.5*(a0 - delta)*sign(y);
end

if (abs(a) <= delta)
	fst = -r*a / delta;
else
	fst = -r*sign(a);
end
u1 = single(x1 + T*x2); %计算跟踪信号
u2 = single(x2 + T*fst); % 计算微分信号

== matlab function THSDemo/NavigationModel/GPSNav/1/GPS_Data_Process/TD_baro/MATLAB Function2 ==
  data: T input single; u1 output; u0 input; u1 input single; u2 input single; h input single; r input single; u2 output
function [u1,u2]=diff_TD_2(T,u0,u1,u2,h,r)
    %init
    %T是信号周期，u0原始信号输入，u1跟踪原始信号，u2原始信号差分值，
    %h滤波因子（h=T时接近一阶差分）越大滤波好延迟大；r速度因子，越大跟踪的越快但是噪声放大；

x1=0; x2=0;
delta=0;
delta0=0;
y=0;
fabs_y=0;
a0=0;
a=0;
fst=0;

x1 = u1;
x2 = u2;
delta = r*h;
delta0 = delta*h;
y = x1 - u0 + h*x2;
fabs_y = abs(y);   
a0 = sqrt(delta*delta + 8 * r*fabs_y);

if (fabs_y <= delta0)
	a = x2 + y / h;
else
    a = x2 + 0.5*(a0 - delta)*sign(y);
end

if (abs(a) <= delta)
	fst = -r*a / delta;
else
	fst = -r*sign(a);
end
u1 = single(x1 + T*x2); %计算跟踪信号
u2 = single(x2 + T*fst); % 计算微分信号
